simulink model "DCServomotorWResLoad_Nominal_Tracking_Quanser"  (R2024b)
settings: Solver=VariableStepAuto  StartTime=0.0  StopTime=4  MaxStep=10e-7  MinStep=10e-9  RelTol=1e-1
undefined symbols (not defined in the file): delta_n, DiscIntNeverNeededParam, K_nom, Nu, Nx, rads2rpm, rpm2rads, sens, wc, wc2
libraries: simulink x1
settings Model: Creator=liliy  LastModifiedBy=lenovo
settings SolverCC: ZeroCrossAlgorithm=Adaptive
settings DataIOCC: ReturnWorkspaceOutputs=off
settings DebuggingCC: IgnoredZcDiagnostic=none

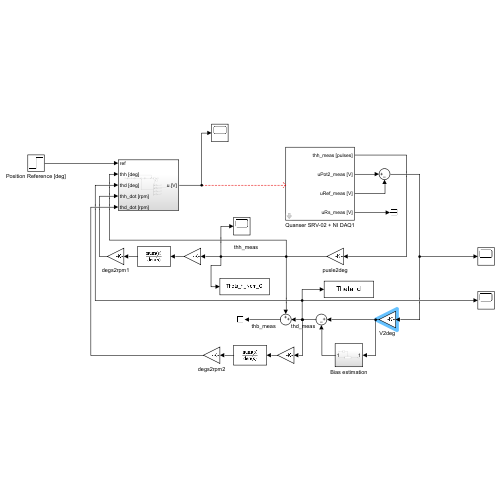
[thumbnail: Simulink's stored preview of the top-level diagram]
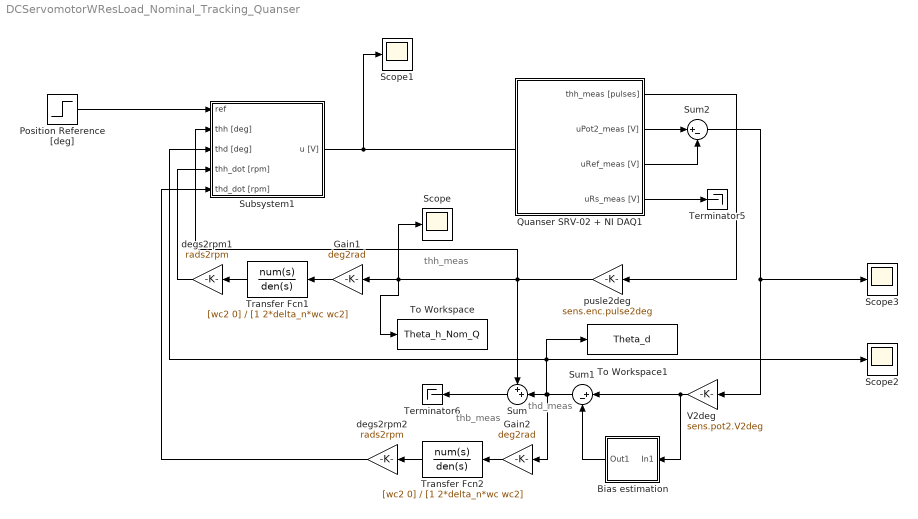
== system DCServomotorWResLoad_Nominal_Tracking_Quanser ==
  note: thh_meas
  note: thd_meas
  note: thb_meas
  Bias estimation : Subsystem
  Gain1 : Gain  Gain=deg2rad
  Gain2 : Gain  Gain=deg2rad
  Position Reference [deg] : Step  After=50  SampleTime=0
  Quanser SRV-02 + NI DAQ1 : Subsystem  mask(Quanser SRV-02 (with resonant load) + NI DAQ){Ts=0.000001, fricType=Coulomb + viscous, lockShaft=on, beamInitPos=15}
      mask prompts: Ts "NI DAQ Sample Time:"; fricType "Friction model"; lockShaft "Lock motor shaft"; beamInitPos "Beam initial position [deg]:"
      mask help: Quanser SRV-02 (with resonant load) + NI DAQ model.
      mask init:
      | %%
      | % Riccardo Antonello (riccardo.antonello@unipd.it)
      | %
      | % April 28, 2020
      | %
      | % Dept. of Information Engineering, University of Padova
      | %
      | 
      | %%  Conversion gains
      | deg2rad = pi/180;                   %   [deg]   -> [rad]
      | rad2deg = 180/pi;                   %   [rad]   -> [deg]
      | 
      | 
      | %%  Sensors data
      | 
      | %   shunt resistor
      | sens.curr.Rs = 0.5;   
      | 
      | %   Hewlett-Packard HEDS-5540#A06 optical encoder
      | sens.enc.ppr = 500*4;                                                   %   pulses per rotation
      | sens.enc.pulse2deg = 360/sens.enc.ppr;                                  %   [pulses] -> [deg]
      | sens.enc.pulse2rad = 2*pi/sens.enc.ppr;                                 %   [pulses] -> [rad]
      | sens.enc.deg2pulse = sens.enc.ppr/360;                                  %   [deg] -> [pulses]
      | sens.enc.rad2pulse = sens.enc.ppr/2/pi;                                 %   [rad] -> [pulses]
      | 
      | %   potentiometer 2 (Spectrol 357-0-0-103) - installed on hub
      | sens.pot2.range.R      = 10e3;                                          %   ohmic value range 
      | sens.pot2.range.V      = 5;                                             %   voltage range
      | sens.pot2.range.th_deg = 340;                                           %   angle range [deg]
      | sens.pot2.range.th     = sens.pot2.range.th_deg * deg2rad;              %   angle range [rad]                           
      | sens.pot2.deg2V        = sens.pot2.range.V / sens.pot2.range.th_deg;    %   sensitivity [V/deg]
      | sens.pot2.rad2V        = sens.pot2.range.V / sens.pot2.range.th;        %   sensitivity [V/rad]
      | sens.pot2.V2deg        = 1/sens.pot2.deg2V;                             %   conversion gain [V] -> [deg]
      | sens.pot2.V2rad        = 1/sens.pot2.rad2V;                             %   conversion gain [V] -> [rad]
      | sens.pot2.noise.var    = 3.5e-7;                                        %   out noise variance [V^2]
      | 
      | 
      | %%  Data acquisition board (daq) data
      | 
      | %   NI PCI-6221 DAC data
      | daq.dac.bits = 16;                                  %   resolution (bits)
      | daq.dac.fs   = 10;                                  %   full scale 
      | daq.dac.q    = 2*daq.dac.fs/(2^daq.dac.bits-1);     %	quantization
      | 
      | %   NI PCI-6221 ADC data
      | daq.adc.bits = 16;                                  %   resolution (bits)
      | daq.adc.fs   = 10;                                  %   full scale (as set in SLDRT Analog Input block)
      | daq.adc.q    = 2*daq.adc.fs/(2^daq.adc.bits-1);     %   quantization   
      | 
      | 
      | %%  Set beam initial position
      | % SRV02Handle = find_system(gcb, ...
      | %     'LookUnderMasks', 'on', ...
      | %     'FindAll', 'on', ...
      | %     'FollowLinks', 'on', ...
      | %     'SearchDepth', '1', ...
      | %     'BlockType', 'ModelReference', ...
      | %     'Name', 'Quanser SRV-02');
      | %
      | % %get_param(SRV02Handle, 'InstanceParameters')
      | % InstanceParams = get_param(SRV02Handle, 'InstanceParameters');
      | % for k = 1:length(InstanceParams)
      | %     if strcmp(InstanceParams(k).Name, 'thb0')
      | %         if lockShaft
      | %             InstanceParams(k).Value = sprintf('%f', beamInitPos);
      | %         else
      | %             InstanceParams(k).Value = sprintf('%f', 0);    
      | %         end
      | %         set_param(SRV02Handle, 'InstanceParameters', InstanceParams);
      | %         break;
      | %     end
      | % end
      | 
      | if lockShaft
      |     thb0 = beamInitPos;
      | else
      |     thb0 = 0;    
      | end
      | 
      | 
      | %%  Mask initialization
      | if lockShaft
      |     
      |     %   find Inport handle
      |     InPortHandle = find_system(gcb, ...
      |         'LookUnderMasks', 'on', ...
      |         'FindAll', 'on', ...
      |         'FollowLinks', 'on', ...
      |         'SearchDepth', '1', ...
      |         'BlockType', 'Inport', ...
      |         'Name', 'u [V]');
      |     
      |     if ~isempty(InPortHandle)
      |     
      |         %   find DAC handle
      |         DACHandle = find_system(gcb, ...
      |             'LookUnderMasks', 'on', ...
      |             'FindAll', 'on', ...
      |             'FollowLinks', 'on', ...
      |             'SearchDepth', '1', ...
      |             'BlockType', 'SubSystem', ...
      |             'Name', 'DAC');  
      | 
      |         %   remove Inport output connection   
      |         InportConn = get_param(InPortHandle, 'PortConnectivity');
      |         delete_line(gcb, InportConn.Position);
      | 
      |         %   remove Inport block
      |         delete_block(InPortHandle);
      | 
      |         %   add Constant block
      |         ConstantHandle = add_block( ...
      |             'simulink/Sources/Constant', [gcb, '/u [V]'], ...
      |             'Position', [20   -37    50   -23], ...
      |             'Value', '0');
      | 
      |         %   connect Constant to DAC block
      |         DACPortHandles = get_param(DACHandle, 'PortHandles');
      |         ConstantPortHandles = get_param(ConstantHandle, 'PortHandles');
      |         add_line(gcb, ConstantPortHandles.Outport(1), DACPortHandles.Inport(1));
      |     
      |     end
      |     
      | else
      |     
      |     %   find Constant handle
      |     ConstantHandle = find_system(gcb, ...
      |         'LookUnderMasks', 'on', ...
      |         'FindAll', 'on', ...
      |         'FollowLinks', 'on', ...
      |         'SearchDepth', '1', ...
      |         'BlockType', 'Constant', ...
      |         'Name', 'u [V]');
      |     
      |     if ~isempty(ConstantHandle)
      |     
      |         %   find DAC handle
      |         DACHandle = find_system(gcb, ...
      |             'LookUnderMasks', 'on', ...
      |             'FindAll', 'on', ...
      |             'FollowLinks', 'on', ...
      |             'SearchDepth', '1', ...
      |             'BlockType', 'SubSystem', ...
      |             'Name', 'DAC');  
      |  
      |         %   remove Constant output connection   
      |         ConstantConn = get_param(ConstantHandle, 'PortConnectivity');
      |         delete_line(gcb, ConstantConn.Position);
      | 
      |         %   remove Inport block
      |         delete_block(ConstantHandle);   
      | 
      |         %   add Inport block
      |         InportHandle = add_block( ...
      |             'simulink/Sources/In1', [gcb, '/u [V]'], ...
      |             'Position', [20   -37    50   -23], ...
      |             'Port', '1');
      | 
      |         %   connect Constant to DAC block
      |         DACPortHandles = get_param(DACHandle, 'PortHandles');
      |         InportPortHandles = get_param(InportHandle, 'PortHandles');
      |         add_line(gcb, InportPortHandles.Outport(1), DACPortHandles.Inport(1));
      |     
      |      end
      |     
      | end
      mask Help:
      | Riccardo Antonello (antonello@dei.unipd.it)
      | 
      | April 28, 2020
      | 
      | Dept. of Information Engineering, University of Padova
      mask TypeOptions fricType: Coulomb + viscous | Karnopp
      mask Callback lockShaft:
      | %   get status of check box
      | lockShaft = get_param(gcb, 'lockShaft');
      | 
      | %   get current value of MaskVisibilities property
      | maskVisibilities = get_param(gcb, 'MaskVisibilities');
      | 
      | %   set visibility of the dialog box element
      | if strcmp(lockShaft, 'on')
      |     maskVisibilities{4} = 'on';
      | else
      |     maskVisibilities{4} = 'off';
      | end
      | 
      | % Set the 'MaskVisibilities' property for each parameter in mask
      | set_param( gcb, 'MaskVisibilities', maskVisibilities);
  Scope{,1..3} (4 alike) : Scope
  Subsystem1 : Subsystem
  Sum : Sum  Inputs=++|
  Sum1 : Sum  Inputs=|+-
  Sum2 : Sum  Inputs=|+-
  Terminator5 : Terminator
  Terminator6 : Terminator
  To Workspace : ToWorkspace  VariableName=Theta_h_Nom_Q  SaveFormat=Structure With Time  SampleTime=-1
  To Workspace1 : ToWorkspace  VariableName=Theta_d  SaveFormat=Structure With Time  SampleTime=-1
  Transfer Fcn1 : TransferFcn  Numerator=[wc2 0]  Denominator=[1 2*delta_n*wc wc2]
  Transfer Fcn2 : TransferFcn  Numerator=[wc2 0]  Denominator=[1 2*delta_n*wc wc2]
  V2deg : Gain  Gain=sens.pot2.V2deg
  degs2rpm1 : Gain  Gain=rads2rpm
  degs2rpm2 : Gain  Gain=rads2rpm
  pusle2deg : Gain  Gain=sens.enc.pulse2deg
  wires:
  Quanser SRV-02 + NI DAQ1/1(thh_meas [pulses]) -> pusle2deg/1
  pusle2deg/1 -> Subsystem1/2(thh [deg]), Gain1/1, To Workspace/1, Scope/1, Sum/1
  Sum/1 -> Terminator6/1
  Subsystem1/1(u [V]) -> Scope1/1
  Quanser SRV-02 + NI DAQ1/4(uRs_meas [V]) -> Terminator5/1
  Quanser SRV-02 + NI DAQ1/3(uRef_meas [V]) -> Sum2/2
  Position Reference [deg]/1 -> Subsystem1/1(ref)
  Gain1/1 -> Transfer Fcn1/1
  Transfer Fcn1/1 -> degs2rpm1/1
  Gain2/1 -> Transfer Fcn2/1
  Transfer Fcn2/1 -> degs2rpm2/1
  degs2rpm2/1 -> Subsystem1/5(thd_dot [rpm])
  degs2rpm1/1 -> Subsystem1/4(thh_dot [rpm])
  Sum1/1 -> Gain2/1, Scope2/1, Subsystem1/3(thd [deg]), To Workspace1/1, Sum/2
  Bias estimation/1(Out1) -> Sum1/2
  V2deg/1 -> Bias estimation/1(In1), Sum1/1
  Quanser SRV-02 + NI DAQ1/2(uPot2_meas [V]) -> Sum2/1
  Sum2/1 -> V2deg/1, Scope3/1

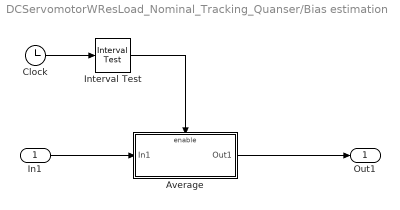
== system DCServomotorWResLoad_Nominal_Tracking_Quanser/Bias estimation ==
  In1 : Inport
  Average : Subsystem  TreatAsAtomicUnit=on
  Clock : Clock
  Interval Test : simulink/Logic and Bit Operations/Interval Test  IntervalClosedRight=on  uplimit=0.2  IntervalClosedLeft=on  lowlimit=0.7  OutDataTypeStr=boolean
  Out1 : Outport
  wires:
  In1/1 -> Average/1(In1)
  Average/1(Out1) -> Out1/1
  Clock/1 -> Interval Test/1
  Interval Test/1 -> Average/Enable

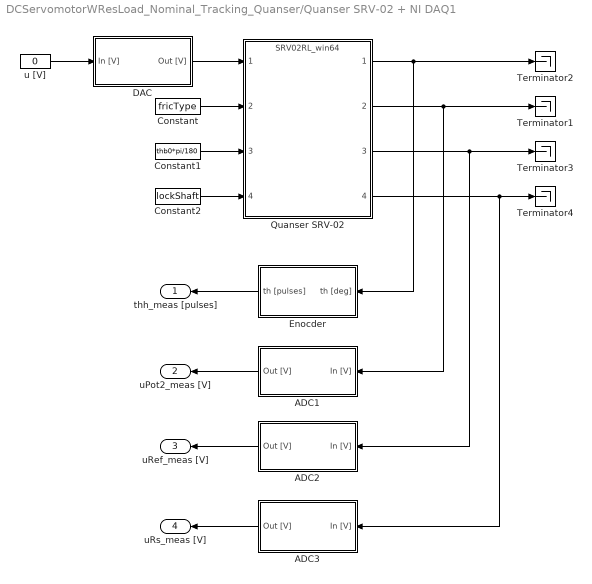
== system DCServomotorWResLoad_Nominal_Tracking_Quanser/Quanser SRV-02 + NI DAQ1 ==
  ADC1 : Subsystem
  ADC2 : Subsystem
  ADC3 : Subsystem
  Constant : Constant  Value=fricType
  Constant1 : Constant  Value=thb0*pi/180  SampleTime=Inf
  Constant2 : Constant  Value=lockShaft  SampleTime=Inf
  DAC : Subsystem
  Enocder : Subsystem
  Quanser SRV-02 : ModelReference  ModelNameDialog=SRV02RL_win64.slxp  ModelReferenceVersion=1.76  CopyOfModelProtected=on
  Terminator{1..4} (4 alike) : Terminator
  u [V] : Constant  Value=0
  thh_meas [pulses] : Outport
  uPot2_meas [V] : Outport  Port=2
  uRef_meas [V] : Outport  Port=3
  uRs_meas [V] : Outport  Port=4
  wires:
  ADC2/1(Out [V]) -> uRef_meas [V]/1
  Quanser SRV-02/4 -> Terminator4/1, ADC3/1(In [V])
  Constant2/1 -> Quanser SRV-02/4
  Constant1/1 -> Quanser SRV-02/3
  ADC1/1(Out [V]) -> uPot2_meas [V]/1
  Quanser SRV-02/3 -> Terminator3/1, ADC2/1(In [V])
  Constant/1 -> Quanser SRV-02/2
  Quanser SRV-02/1 -> Enocder/1(th [deg]), Terminator2/1
  Quanser SRV-02/2 -> Terminator1/1, ADC1/1(In [V])
  DAC/1(Out [V]) -> Quanser SRV-02/1
  ADC3/1(Out [V]) -> uRs_meas [V]/1
  Enocder/1(th [pulses]) -> thh_meas [pulses]/1
  u [V]/1 -> DAC/1(In [V])

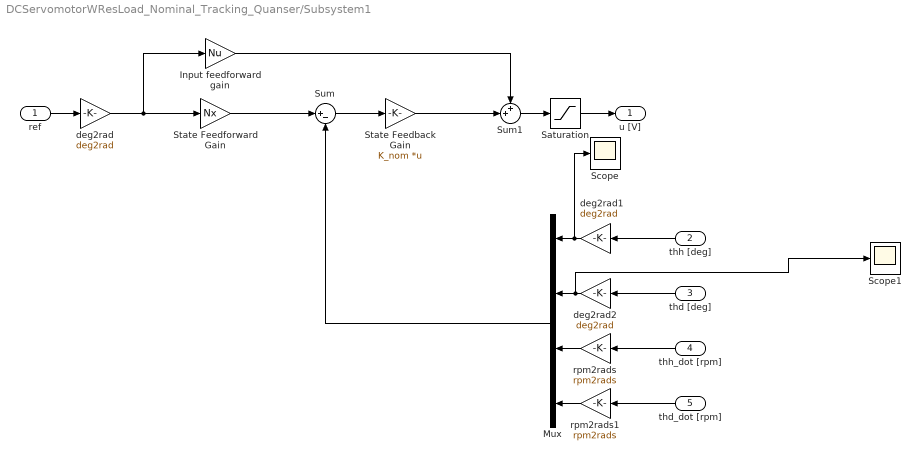
== system DCServomotorWResLoad_Nominal_Tracking_Quanser/Subsystem1 ==
  ref : Inport
  thh [deg] : Inport  Port=2
  thd [deg] : Inport  Port=3
  thh_dot [rpm] : Inport  Port=4
  thd_dot [rpm] : Inport  Port=5
  Input feedforward gain : Gain  Gain=Nu
  Mux : Mux
  Saturation : Saturate  UpperLimit=12  LowerLimit=-12
  Scope : Scope
  Scope1 : Scope
  State Feedback Gain : Gain  Gain=K_nom  Multiplication=Matrix(K*u)
  State Feedforward Gain : Gain  Gain=Nx
  Sum : Sum  Inputs=|+-
  Sum1 : Sum  Inputs=++|
  deg2rad : Gain  Gain=deg2rad
  deg2rad1 : Gain  Gain=deg2rad
  deg2rad2 : Gain  Gain=deg2rad
  rpm2rads : Gain  Gain=rpm2rads
  rpm2rads1 : Gain  Gain=rpm2rads
  u [V] : Outport
  wires:
  ref/1 -> deg2rad/1
  deg2rad/1 -> Input feedforward gain/1, State Feedforward Gain/1
  State Feedforward Gain/1 -> Sum/1
  Sum/1 -> State Feedback Gain/1
  State Feedback Gain/1 -> Sum1/2
  Input feedforward gain/1 -> Sum1/1
  Sum1/1 -> Saturation/1
  Mux/1 -> Sum/2
  deg2rad1/1 -> Scope/1, Mux/1
  thh [deg]/1 -> deg2rad1/1
  deg2rad2/1 -> Scope1/1, Mux/2
  thd [deg]/1 -> deg2rad2/1
  thh_dot [rpm]/1 -> rpm2rads/1
  rpm2rads/1 -> Mux/3
  rpm2rads1/1 -> Mux/4
  thd_dot [rpm]/1 -> rpm2rads1/1
  Saturation/1 -> u [V]/1

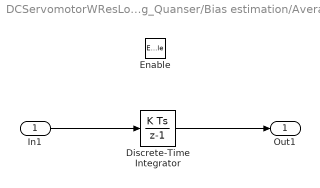
== system DCServomotorWResLoad_Nominal_Tracking_Quanser/Bias estimation/Average ==
  In1 : Inport
  Enable : EnablePort
  Discrete-Time Integrator : DiscreteIntegrator  SampleTime=-1  ICPrevOutput=DiscIntNeverNeededParam  ICPrevScaledInput=DiscIntNeverNeededParam
  Out1 : Outport
  wires:
  In1/1 -> Discrete-Time Integrator/1
  Discrete-Time Integrator/1 -> Out1/1

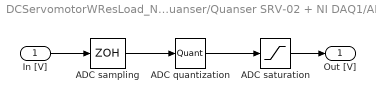
== system DCServomotorWResLoad_Nominal_Tracking_Quanser/Quanser SRV-02 + NI DAQ1/ADC1 ==
  In [V] : Inport
  ADC quantization : Quantizer  QuantizationInterval=daq.adc.q
  ADC sampling : ZeroOrderHold  SampleTime=Ts
  ADC saturation : Saturate  UpperLimit=daq.adc.fs  LowerLimit=-daq.adc.fs
  Out [V] : Outport
  wires:
  ADC quantization/1 -> ADC saturation/1
  In [V]/1 -> ADC sampling/1
  ADC sampling/1 -> ADC quantization/1
  ADC saturation/1 -> Out [V]/1

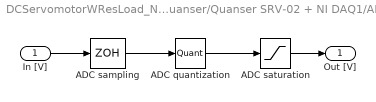
== system DCServomotorWResLoad_Nominal_Tracking_Quanser/Quanser SRV-02 + NI DAQ1/ADC2 ==
  In [V] : Inport
  ADC quantization : Quantizer  QuantizationInterval=daq.adc.q
  ADC sampling : ZeroOrderHold  SampleTime=Ts
  ADC saturation : Saturate  UpperLimit=daq.adc.fs  LowerLimit=-daq.adc.fs
  Out [V] : Outport
  wires:
  ADC saturation/1 -> Out [V]/1
  ADC sampling/1 -> ADC quantization/1
  In [V]/1 -> ADC sampling/1
  ADC quantization/1 -> ADC saturation/1

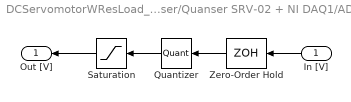
== system DCServomotorWResLoad_Nominal_Tracking_Quanser/Quanser SRV-02 + NI DAQ1/ADC3 ==
  In [V] : Inport
  Quantizer : Quantizer  QuantizationInterval=daq.adc.q
  Saturation : Saturate  UpperLimit=daq.adc.fs  LowerLimit=-daq.adc.fs
  Zero-Order Hold : ZeroOrderHold  SampleTime=Ts
  Out [V] : Outport
  wires:
  Zero-Order Hold/1 -> Quantizer/1
  Quantizer/1 -> Saturation/1
  In [V]/1 -> Zero-Order Hold/1
  Saturation/1 -> Out [V]/1

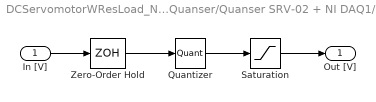
== system DCServomotorWResLoad_Nominal_Tracking_Quanser/Quanser SRV-02 + NI DAQ1/DAC ==
  In [V] : Inport
  Quantizer : Quantizer  QuantizationInterval=daq.dac.q
  Saturation : Saturate  UpperLimit=daq.dac.fs  LowerLimit=-daq.dac.fs
  Zero-Order Hold : ZeroOrderHold  SampleTime=Ts
  Out [V] : Outport
  wires:
  Saturation/1 -> Out [V]/1
  Zero-Order Hold/1 -> Quantizer/1
  In [V]/1 -> Zero-Order Hold/1
  Quantizer/1 -> Saturation/1

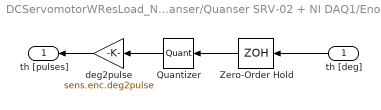
== system DCServomotorWResLoad_Nominal_Tracking_Quanser/Quanser SRV-02 + NI DAQ1/Enocder ==
  th [deg] : Inport
  Quantizer : Quantizer  QuantizationInterval=sens.enc.pulse2deg
  Zero-Order Hold : ZeroOrderHold  SampleTime=Ts
  deg2pulse : Gain  Gain=sens.enc.deg2pulse
  th [pulses] : Outport
  wires:
  deg2pulse/1 -> th [pulses]/1
  Zero-Order Hold/1 -> Quantizer/1
  th [deg]/1 -> Zero-Order Hold/1
  Quantizer/1 -> deg2pulse/1
